simulink model "emso2"  (Simulink 7.1)
settings: Solver=ode45  StartTime=0.0  StopTime=10  RelTol=1e-3
settings Model: Creator=lades  LastModifiedBy=Administrator
settings DataIOCC: ExternalInput=Az

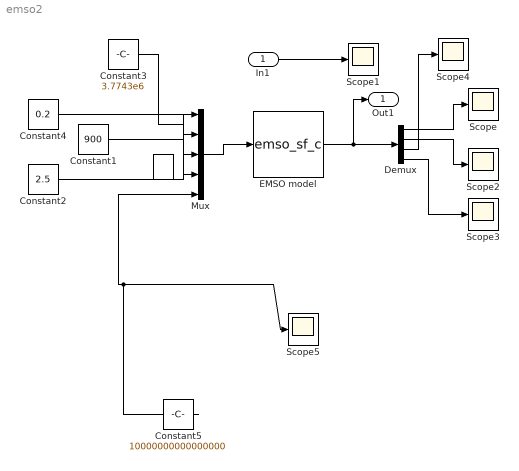
== system emso2 ==
  In1 : Inport  OutDataType=sfix(16)  OutScaling=2^0
  Constant1 : Constant  Value=900  OutDataType=sfix(16)  OutScaling=2^0
  Constant2 : Constant  Value=2.5  OutDataType=sfix(16)  OutScaling=2^0
  Constant3 : Constant  Value=3.7743e6  OutDataType=sfix(16)  OutScaling=2^0
  Constant4 : Constant  Value=0.2  OutDataType=sfix(16)  OutScaling=2^0
  Constant5 : Constant  Value=10000000000000000  OutDataType=sfix(16)  OutScaling=2^0
  Demux : Demux
  EMSO model : S-Function  FunctionName=emso_sf_c  Parameters='batch_dist.ems',5,4  EnableBusSupport=off
  Mux : Mux  Inputs=5
  Scope{,1..5} (6 alike) : Scope
      Scope settings: TimeRange=2  YMin=294.46  YMax=294.505
      Scope2 settings: TimeRange=2  YMin=0.792305  YMax=0.79233  SaveName=ScopeData2
      Scope3 settings: TimeRange=15  YMin=2.25  YMax=2.5  SaveName=ScopeData3
      Scope4 settings: TimeRange=2  YMin=0.20736  YMax=0.207415  SaveName=ScopeData4
      Scope5 settings: TimeRange=15  YMin=2.25  YMax=2.5  SaveName=ScopeData5
  Out1 : Outport  OutDataType=sfix(16)  OutScaling=2^0
  wires:
  EMSO model/1 -> Out1/1, Demux/1
  In1/1 -> Scope1/1
  Constant3/1 -> Mux/1
  Mux/1 -> EMSO model/1
  Demux/4 -> Scope3/1
  Demux/3 -> Scope4/1
  Demux/2 -> Scope2/1
  Demux/1 -> Scope/1
  Constant1/1 -> Mux/2
  Constant2/1 -> Mux/3
  Constant4/1 -> Mux/4
  Constant5/1 -> Scope5/1, Mux/5
